simulink model "ZF02HD250606_23a"  (R2023a)
settings: Solver=ode4  StartTime=0.0  StopTime=inf  FixedStep=0.002  RelTol=1e-3
InitFcn:
  |  T_c = 0.002;
undefined symbols (not defined in the file): DiscIntNeverNeededParam, Discrete, magnitude, Time
libraries: AFCToolbox x33, simulink x28, simulink_extras x7, sharedtransform x2, ctrlSharedLib x2, aerolibconvert2 x1, aerolibtransform2 x1, dspstat3 x1, dspsolvers x1
(part 3 of 3)

== matlab function ZF02HD250606_23a/BasicModel/AttiAltHold/h_fusion1/MATLAB Function ==
  data: nonod_sts input; fusedHeight output; H input; gps_NEG_h input
function fusedHeight = HeightFusedAlg(nonod_sts, H, gps_NEG_h)
    persistent prev_nonod_sts prev_fused_height transition_counter transition_duration
    % 初始化持久变量
    if isempty(transition_counter)
        transition_counter = 0;
        prev_nonod_sts = nonod_sts; % 初始化前一个状态
        prev_fused_height = H; % 初始化前一个融合高度，这里假设初始为气压高度
        transition_duration = 10; % 假设过渡持续10次调用
    end
    
    % 根据nonod_sts状态确定gpsWeight
    gpsWeight = getGpsWeight(nonod_sts);
    pressureWeight = 1 - gpsWeight;

     % 融合高度计算, 注意：因为GPS高度是北东地坐标系下参数，其值为负，所以在加权平均时要取反
    tmpFusedHeight = (pressureWeight * H) + (gpsWeight * (-gps_NEG_h));

    % 检测状态是否发生改变
    if nonod_sts ~= prev_nonod_sts
        % 重置平滑处理计数器
        transition_counter = 0;
        prev_nonod_sts = nonod_sts; % 更新前一个状态
    end

    % 状态切换过程中的平滑处理
    if transition_counter < transition_duration
        % 状态改变，平滑过渡
        % 逐步改变输出高度，从切换点的高度过渡到新的状态高度
        fusedHeight = lerp(prev_fused_height, tmpFusedHeight, transition_counter / transition_duration);
        % 更新平滑处理计数器
        transition_counter = transition_counter + 1;
    else
        % 状态稳定，直接使用确定权重
        transition_counter = transition_duration; % 保持计数器在最大值，避免无限增长
            % 保存当前融合高度，用于下一次调用
        prev_fused_height = tmpFusedHeight;

    % 返回融合后的高度
        fusedHeight = tmpFusedHeight;
    end  
end

% 辅助函数：线性插值
function value = lerp(a, b, t)
    value = a + (b - a) * t;
end

% 根据前一个nanoD状态确定初始的gpsWeight
function gpsWeight = getGpsWeight(nonod_sts)
    switch nonod_sts
        case 1
            gpsWeight = 0.1;
        case 4
            gpsWeight = 1;
        otherwise
            gpsWeight = 0;
    end
end

== matlab function ZF02HD250606_23a/BasicModel/AttiAltHold/ReturnShutOff/MATLAB Function ==
  data: returnFlg input; height input; flag output
function flag = detectHeight(returnFlg,height)
    persistent count;  % 创建一个持久变量来存储计数值
    persistent locked; % 创建一个持久变量来存储锁定状态

    if returnFlg
        % 检测高度是否小于30, 锁定条件为最小次数200
        minH = 30;  minCount = 200;
    
        % 初始化计数值和锁定状态
        if isempty(count)
            count = 0;
            locked = 0;
        end
    
        % 检测高度是否小于30
        if height < minH
            count = count + 1; % 如果高度小于30，计数值加1
        else
            count = 0;         % 否则，计数值清0
        end
    
        % 检测是否达到锁定条件
        if count > minCount && ~locked
            locked = 1;       % 如果计数值大于500且未锁定，则锁定状态
        end
    
        % 输出锁定状态或当前计数值
        if locked
            flag = 1;         % 如果已锁定，始终输出1
        else
            flag = 0;         % 否则，输出0
        end
    else
        flag = 0;            % 非自主降落阶段为0
    end
end

== matlab function ZF02HD250606_23a/NavigationModel/GPSNav/1/GPS_Data_Process/LLA2NED/initGPSLLA ==
  data: QGCinitflag input; gpsLLA0_rad output; GPSfixtype input; gps_LLA_rad input; init_GPSLLAflag output; GPSHdop input
function [gpsLLA0_rad,init_GPSLLAflag] = initGPSLLA0(QGCinitflag,GPSfixtype,gps_LLA_rad,GPSHdop)
    persistent initGPSLLAflag;
    persistent gpsLLA0;

    if isempty(initGPSLLAflag)
        initGPSLLAflag = 0;
    end
    if isempty(gpsLLA0)
        %初始GPS未进入定位状态，给定值
%          gpsLLA0 = [28.2/57.3;113/57.3;0];
        gpsLLA0 = zeros(3,1);
    end
    %if (initGPSLLAflag == 0 && GPSfixtype >= 3 && GPSHdop <= 2) || (QGCinitflag == 1 && GPSfixtype >= 3)
    if (initGPSLLAflag == 0 && GPSfixtype >= 1 && GPSHdop <= 5) || (QGCinitflag == 1 && GPSfixtype >= 1)
        % 当GPS第一次初始化位置时，当GPSfixtype >=1 时，自动初始化一次位置，initGPSLLAflag置1
        % 或者是利用QGCinitflag地面站重新修正，不过需要满足GPSfixtype>=1的条件
        gpsLLA0 = gps_LLA_rad;
        initGPSLLAflag = 1;
    end
    gpsLLA0_rad = gpsLLA0;
    init_GPSLLAflag = initGPSLLAflag;
end

== matlab function ZF02HD250606_23a/NavigationModel/GPSNav/1/GPS_Data_Process/TD_baro1/MATLAB Function2 ==
  data: T input single; u1 output; u0 input; u1 input single; u2 input single; h input single; r input single; u2 output
function [u1,u2]=diff_TD_2(T,u0,u1,u2,h,r)
    %init
    %T是信号周期，u0原始信号输入，u1跟踪原始信号，u2原始信号差分值，
    %h滤波因子（h=T时接近一阶差分）越大滤波好延迟大；r速度因子，越大跟踪的越快但是噪声放大；

x1=0; x2=0;
delta=0;
delta0=0;
y=0;
fabs_y=0;
a0=0;
a=0;
fst=0;

x1 = u1;
x2 = u2;
delta = r*h;
delta0 = delta*h;
y = x1 - u0 + h*x2;
fabs_y = abs(y);   
a0 = sqrt(delta*delta + 8 * r*fabs_y);

if (fabs_y <= delta0)
	a = x2 + y / h;
else
    a = x2 + 0.5*(a0 - delta)*sign(y);
end

if (abs(a) <= delta)
	fst = -r*a / delta;
else
	fst = -r*sign(a);
end
u1 = single(x1 + T*x2); %计算跟踪信号
u2 = single(x2 + T*fst); % 计算微分信号

== matlab function ZF02HD250606_23a/NavigationModel/GPSNav/1/GPS_Data_Process/TD_baro/MATLAB Function2 ==
  data: T input single; u1 output; u0 input; u1 input single; u2 input single; h input single; r input single; u2 output
function [u1,u2]=diff_TD_2(T,u0,u1,u2,h,r)
    %init
    %T是信号周期，u0原始信号输入，u1跟踪原始信号，u2原始信号差分值，
    %h滤波因子（h=T时接近一阶差分）越大滤波好延迟大；r速度因子，越大跟踪的越快但是噪声放大；

x1=0; x2=0;
delta=0;
delta0=0;
y=0;
fabs_y=0;
a0=0;
a=0;
fst=0;

x1 = u1;
x2 = u2;
delta = r*h;
delta0 = delta*h;
y = x1 - u0 + h*x2;
fabs_y = abs(y);   
a0 = sqrt(delta*delta + 8 * r*fabs_y);

if (fabs_y <= delta0)
	a = x2 + y / h;
else
    a = x2 + 0.5*(a0 - delta)*sign(y);
end

if (abs(a) <= delta)
	fst = -r*a / delta;
else
	fst = -r*sign(a);
end
u1 = single(x1 + T*x2); %计算跟踪信号
u2 = single(x2 + T*fst); % 计算微分信号
